simulink model "cornering_simulation_self_contained"  (R2026a)
settings: Solver=VariableStepAuto
settings Model: Creator=mattr  LastModifiedBy=mattr

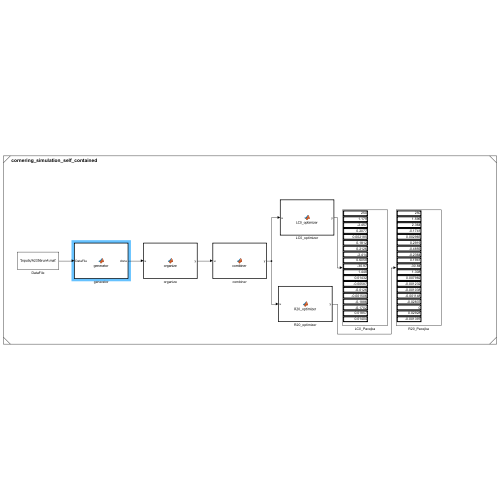
[thumbnail: Simulink's stored preview of the top-level diagram]
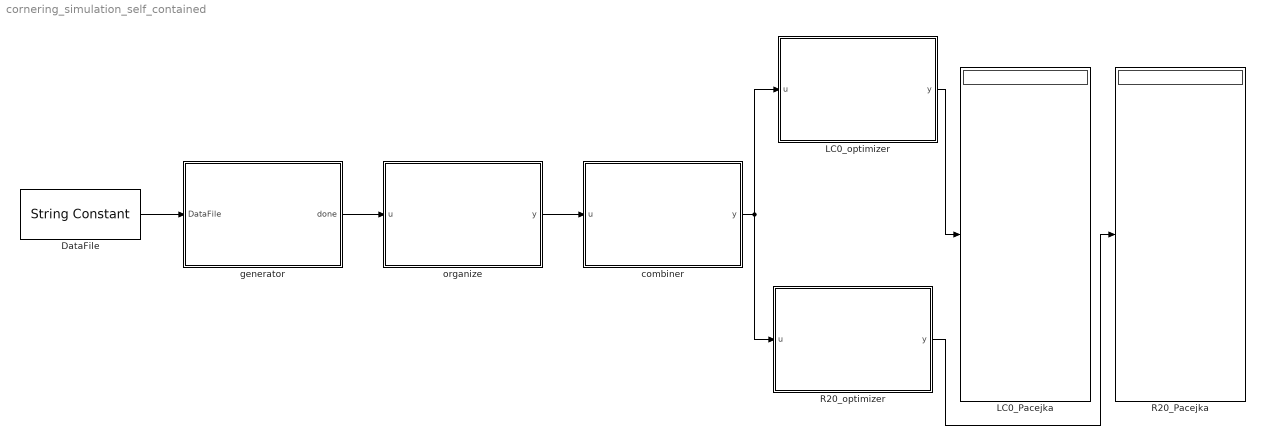
== system cornering_simulation_self_contained ==
  DataFile : StringConstant  String='Inputs/A2356run4.mat'
  LC0_Pacejka : Display
  LC0_optimizer : MATLAB Function  TreatAsAtomicUnit=on
  R20_Pacejka : Display
  R20_optimizer : MATLAB Function  TreatAsAtomicUnit=on
  combiner : MATLAB Function  TreatAsAtomicUnit=on
  generator : MATLAB Function  TreatAsAtomicUnit=on
  organize : MATLAB Function  TreatAsAtomicUnit=on
  wires:
  organize/1(y) -> combiner/1(u)
  combiner/1(y) -> R20_optimizer/1(u), LC0_optimizer/1(u)
  generator/1(done) -> organize/1(u)
  R20_optimizer/1(y) -> R20_Pacejka/1
  LC0_optimizer/1(y) -> LC0_Pacejka/1
  DataFile/1 -> generator/1(DataFile)

== matlab function cornering_simulation_self_contained/generator ==
  data: DataFile input; done output
function done = generator(DataFile)
    coder.extrinsic('evalin', 'assignin', 'disp');
    
    done = 0;
    persistent hasExecuted;
    if isempty(hasExecuted)
        hasExecuted = false;
    end
    
    if ~hasExecuted
        if isstring(DataFile)
            dataFileStr = char(DataFile);
        elseif ischar(DataFile)
            dataFileStr = DataFile;
        else
            dataFileStr = char(DataFile(:)');
        end
        
        assignin('base', 'gen_dataFileStr', dataFileStr);
        evalin('base', [ ...
            'outputFolder = ''data/Outputs/R20Round4&5''; ' ...
            'if ~exist(outputFolder, ''dir''), mkdir(outputFolder); end; ' ...
            'curFile = load(gen_dataFileStr); ' ...
            'disp(["Loaded " gen_dataFileStr]); ' ...
            'runTable = table(curFile.AMBTMP, curFile.ET, curFile.FX, curFile.FY, curFile.FZ, curFile.IA, curFile.MX, curFile.MZ, ' ...
            'curFile.N, curFile.NFX, curFile.NFY, curFile.P, curFile.RE, curFile.RL, curFile.RST, ' ...
            'curFile.SA, curFile.SL, curFile.SR, curFile.TSTC, curFile.TSTI, curFile.TSTO, curFile.V, ' ...
            '''VariableNames'', {''AmbientRoomTemperature'', ''ElapsedTime'', ''LongitudinalForce'', ''LateralForce'', ' ...
            '''NormalForce'', ''InclinationAngle'', ''OverturningMoment'', ''AligningTorque'', ''WheelRotationalSpeed'', ' ...
            '''NormalizedLongitudinalForce_FX_FZ'', ''NormalizedLateralForce_FY_FZ'', ''TirePressure'', ' ...
            '''EffectiveRadius'', ''LoadedRadius'', ''RoadSurfaceTemperature'', ''SlipAngle'', ''SlipRatioTextbook'', ' ...
            '''SlipRatioBasedOnRL'', ''TireSurfaceTemperature_Center'', ''TireSurfaceTemperature_Inboard'', ' ...
            '''TireSurfaceTemperature_Outboard'', ''RoadSpeed''}); ' ...
            'runTable.testid = repmat(string(curFile.testid), height(runTable), 1); ' ...
            'runTable.tireid = repmat(string(curFile.tireid), height(runTable), 1); ' ...
            'runTable.Index = (1:height(runTable))''; ' ...
            'nRows = height(runTable); ' ...
            'subTables = struct(); ' ...
            'subTables.FZ50  = runTable(5006:min(6220, nRows), :); ' ...
            'subTables.FZ100 = runTable(7491:min(8645, nRows), :); ' ...
            'subTables.FZ150 = runTable(3754:min(4937, nRows), :); ' ...
            'subTables.FZ200 = runTable(2546:min(3667, nRows), :); ' ...
            'subTables.FZ250 = [runTable(1:min(2484, nRows), :); runTable(6255:min(7418, nRows), :)]; ' ...
            'outNames = fieldnames(subTables); ' ...
            'for i = 1:numel(outNames) ' ...
            '    fname = fullfile(outputFolder, sprintf("R20_FZ_%s.csv", outNames{i}(3:end))); ' ...
            '    writetable(subTables.(outNames{i}), fname); ' ...
            '    disp(["Saved: " fname]); ' ...
            'end; ' ...
            'disp("All FZ bin CSV files successfully exported.");' ...
        ]);
        
        hasExecuted = true;
    end
    
    done = 1;
end

%% Here is the code as it should be commented above

% function generator()
%
%dataFile     = 'Inputs/A2356run4.mat';     % Change this to round you want
%outputFolder = 'data/Outputs/R20Round4&5'; % Change this to output you want
%
%%% Ensure the output folder exists
%if ~exist(outputFolder, 'dir')
%    mkdir(outputFolder)
%end
%
%% Change these based off of inclination angle/tire type (see Teams)
%idxRange50   = 5006:6220;
%idxRange100  = 7491:8645;
%idxRange150  = 3754:4937;
%idxRange200  = 2546:3667;
%idxRange250a = 1:2484;
%idxRange250b = 6255:7418;

%curFile = load(dataFile);
%disp("Loaded " + dataFile);

%%% Create the table and give names to each of the variables
%runTable = table(curFile.AMBTMP, curFile.ET, curFile.FX, curFile.FY, curFile.FZ, curFile.IA, curFile.MX, curFile.MZ, ...
%    curFile.N, curFile.NFX, curFile.NFY, curFile.P, curFile.RE, curFile.RL, curFile.RST, ...
%    curFile.SA, curFile.SL, curFile.SR, curFile.TSTC, curFile.TSTI, curFile.TSTO, curFile.V, ...
%    'VariableNames', {'AmbientRoomTemperature', 'ElapsedTime', 'LongitudinalForce', 'LateralForce', ...
%    'NormalForce', 'InclinationAngle', 'OverturningMoment', 'AligningTorque', 'WheelRotationalSpeed', ...
%    'NormalizedLongitudinalForce(FX/FZ)', 'NormalizedLateralForce(FY/FZ)', 'TirePressure', ...
%    'EffectiveRadius', 'LoadedRadius', 'RoadSurfaceTemperature', 'SlipAngle', 'SlipRatioTextbook', ...
%    'SlipRatioBasedOnRL', 'TireSurfaceTemperature-Center', 'TireSurfaceTemperature-Inboard', ...
%    'TireSurfaceTemperature-Outboard', 'RoadSpeed'});


%%% Ensure every row has the testid and tireid 
%runTable.testid = repmat(string(curFile.testid), height(runTable), 1);
%runTable.tireid = repmat(string(curFile.tireid), height(runTable), 1);

%%% Index column updated to count up by row starting at 1
%runTable.Index = (1:height(runTable))';

%disp("Run table created with " + height(runTable) + " rows.");

%subTables = struct();

%%% Extracts sub tables from runTable based on the ranges set above
%subTables.FZ50  = runTable(idxRange50,  :);
%subTables.FZ100 = runTable(idxRange100, :);
%subTables.FZ150 = runTable(idxRange150, :);
%subTables.FZ200 = runTable(idxRange200, :);
%subTables.FZ250 = [runTable(idxRange250a, :); runTable(idxRange250b, :)];

%%% Names of all of the FZs 
%outNames = fieldnames(subTables);

%%% Generate output files into the output folder with a naming scheme
%for i = 1:numel(outNames)
%    fname = fullfile(outputFolder, sprintf("R20_FZ_%s.csv", outNames{i}(3:end))); % Change this for tire type/inclination angle
%    writetable(subTables.(outNames{i}), fname);
%    disp("Saved: " + fname);
%end

%disp("All FZ bin CSV files successfully exported.");

%end

== matlab function cornering_simulation_self_contained/combiner ==
  data: u input; y output
function y = combiner(u)
    coder.extrinsic('evalin', 'disp');
    
    y = 0;
    persistent hasExecuted;
    if isempty(hasExecuted)
        hasExecuted = false;
    end
    
    if (u > 0)
        if ~hasExecuted
            evalin('base', [ ...
                'dataFolder = ''data/Outputs/R20Round4&5''; ' ...
                'filteredFiles = dir(fullfile(dataFolder, ''*_filtered.csv'')); ' ...
                'combinedTable = table(); ' ...
                'for i = 1:numel(filteredFiles) ' ...
                '    if contains(filteredFiles(i).name, "combined"), continue; end; ' ...
                '    curFile = fullfile(filteredFiles(i).folder, filteredFiles(i).name); ' ...
                '    disp(["Adding " filteredFiles(i).name]); ' ...
                '    tempTable = readtable(curFile); ' ...
                '    [~, name, ~] = fileparts(filteredFiles(i).name); ' ...
                '    tempTable.SourceFile = repmat({name}, height(tempTable), 1); ' ...
                '    combinedTable = [combinedTable; tempTable]; ' ...
                'end; ' ...
                'combinedTable = sortrows(combinedTable, ''NormalForce''); ' ...
                'outPath = fullfile(dataFolder, ''R20_combined_filtered.csv''); ' ...
                'writetable(combinedTable, outPath); ' ...
                'disp(["Combined filtered data saved as: " outPath]);' ...
            ]);
            hasExecuted = true;
        end
        y = 1;
    end
end

%% Here is the code as it should be commented 

%function combiner()
% 
%     dataFolder = 'data/Outputs/R20Round4&5';
% 
%     %% All of the files from organize.m
%     filteredFiles = dir(fullfile(dataFolder, '*_filtered.csv'));
% 
%     combinedTable = table();
% 
%     for i = 1:numel(filteredFiles)
%         curFile = fullfile(filteredFiles(i).folder, filteredFiles(i).name);
%         disp("Adding " + filteredFiles(i).name);
% 
%         tempTable = readtable(curFile);
% 
%         [~, name, ~] = fileparts(filteredFiles(i).name);
%         tempTable.SourceFile = repmat({name}, height(tempTable), 1);
% 
%         combinedTable = [combinedTable; tempTable];
%     end
% 
%     combinedTable = sortrows(combinedTable, 'NormalForce');
% 
%     outPath = fullfile(dataFolder, 'R20_combined_filtered.csv');
%     writetable(combinedTable, outPath);
% 
%     disp("Combined filtered data saved as: " + outPath);
% 
% 
% end

== matlab function cornering_simulation_self_contained/LC0_optimizer ==
  data: u input; y output size=[19 1]
function y = LC0_optimizer(u)
    coder.extrinsic('evalin', 'disp');
    
    y = zeros(19, 1);
    
    persistent hasExecuted;
    if isempty(hasExecuted)
        hasExecuted = false;
    end
    
    if (u > 0)
        if ~hasExecuted
            evalin('base', [ ...
                'pacejka_calc = @(P, L, FZ, IA, alpha) (' ...
                '    (FZ .* (P(3) + P(4) * ((FZ - P(1)) / P(1))) .* (1 - P(5) * IA.^2) * L(1)) .* ' ...
                '    sin((P(2) * L(2)) * atan(' ...
                '        (((P(10) * P(1) * sin(2 * atan(FZ / (P(11) * P(1) * L(3))))) .* (1 - P(12) * abs(IA)) * L(4) * L(5)) ./ ' ...
                '        ((P(2) * L(2)) * (FZ .* (P(3) + P(4) * ((FZ - P(1)) / P(1))) .* (1 - P(5) * IA.^2) * L(1)))) .* ' ...
                '        (alpha + (P(13) + P(14) * ((FZ - P(1)) / P(1)) + P(15) * IA) * L(6)) - ' ...
                '        ((P(6) + P(7) * ((FZ - P(1)) / P(1))) .* (1 - (P(8) + P(9) * IA) .* sign(alpha)) * L(7)) .* ' ...
                '        (' ...
                '            (((P(10) * P(1) * sin(2 * atan(FZ / (P(11) * P(1) * L(3))))) .* (1 - P(12) * abs(IA)) * L(4) * L(5)) ./ ' ...
                '            ((P(2) * L(2)) * (FZ .* (P(3) + P(4) * ((FZ - P(1)) / P(1))) .* (1 - P(5) * IA.^2) * L(1)))) .* ' ...
                '            (alpha + (P(13) + P(14) * ((FZ - P(1)) / P(1)) + P(15) * IA) * L(6)) - ' ...
                '            atan(' ...
                '                (((P(10) * P(1) * sin(2 * atan(FZ / (P(11) * P(1) * L(3))))) .* (1 - P(12) * abs(IA)) * L(4) * L(5)) ./ ' ...
                '                ((P(2) * L(2)) * (FZ .* (P(3) + P(4) * ((FZ - P(1)) / P(1))) .* (1 - P(5) * IA.^2) * L(1)))) .* ' ...
                '                (alpha + (P(13) + P(14) * ((FZ - P(1)) / P(1)) + P(15) * IA) * L(6))' ...
                '            )' ...
                '        )' ...
                '    )) + FZ .* (P(16) + P(17) * ((FZ - P(1)) / P(1)) + (P(18) + P(19) * ((FZ - P(1)) / P(1))) .* IA) * L(8) * L(5)' ...
                '); ' ...
                'files = {''data/LC0_combined_filtered.csv'', ''data/LC0_IA-2_combined_filtered.csv'', ''data/LC0_IA-4_combined_filtered.csv''}; ' ...
                'validFiles = files(cellfun(@(f) exist(f, ''file'') > 0, files)); ' ...
                'if isempty(validFiles), disp(''Warning: LC0 CSV input files not found. Returning baseline P0.''); LC0_opt_y = [250, 1.17858, -2.45689, 0.207723, 0.00218554, 0.181269, 0.212474, -2.41388, 0.605724, -30.9683, 1.44763, 0.0143188, -0.00587066, -0.0126017, -0.00150596, -0.18861, -0.170156, 0.0185739, 0.0140275]''; else ' ...
                'data = []; for k = 1:numel(validFiles), data = [data; readtable(validFiles{k})]; end; ' ...
                'IA = data.InclinationAngle; FZRaw = data.NormalForce; alpha = data.SlipAngle; FYExperimental = data.LateralForce; source = data.SourceFile; ' ...
                'FZBins = [50, 100, 150, 200, 250]; FYAll = []; FZAll = []; alphaAll = []; IAAll = []; ' ...
                'for i = 1:numel(FZBins), baseTag = sprintf(''LC0_FZ_%d'', FZBins(i)); idx = contains(source, [baseTag ''_filtered'']) | contains(source, [baseTag ''_IA-2_filtered'']) | contains(source, [baseTag ''_IA-4_filtered'']); FYAll = [FYAll; FYExperimental(idx)]; FZAll = [FZAll; FZBins(i) * ones(sum(idx),1)]; alphaAll = [alphaAll; alpha(idx)]; IAAll = [IAAll; IA(idx)]; end; ' ...
                'alphaAll = deg2rad(alphaAll); ' ...
                'P0 = [250, 1.17858, -2.45689, 0.207723, 0.00218554, 0.181269, 0.212474, -2.41388, 0.605724, -30.9683, 1.44763, 0.0143188, -0.00587066, -0.0126017, -0.00150596, -0.18861, -0.170156, 0.0185739, 0.0140275]; ' ...
                'L = ones(1,8); ' ...
                'w_vec = zeros(size(IAAll)); IAvals = unique(IAAll); ' ...
                'for k = 1:numel(IAvals), idx = (IAAll == IAvals(k)); w_vec(idx) = 1 / max(sum(idx), 1); end; ' ...
                'options = optimoptions(''lsqnonlin'', ''Display'', ''iter'', ''MaxFunctionEvaluations'', 20000, ''TolFun'', 1e-8, ''TolX'', 1e-8); ' ...
                'lb = -Inf(1,19); ub = Inf(1,19); lb(1) = 250; ub(1) = 250; ' ...
                'POptimization = lsqnonlin(@(P) w_vec .* (pacejka_calc(P, L, FZAll, IAAll, alphaAll) - FYAll), P0, lb, ub, options); ' ...
                'LC0_opt_y = POptimization(:); disp(''LC0 Optimized Parameters:''); disp(LC0_opt_y); ' ...
                'IAValues = unique(IAAll); colors = lines(numel(FZBins)); ' ...
                'for k = 1:numel(IAValues) ' ...
                '    thisIA = IAValues(k); fig = figure(''Name'', sprintf(''LC0 Pacejka Fit - IA = %.1f deg'', thisIA), ''Visible'', ''on''); hold on; grid on; ' ...
                '    idxIA = (IAAll == thisIA); ' ...
                '    for i = 1:numel(FZBins) ' ...
                '        idx = idxIA & (FZAll == FZBins(i)); ' ...
                '        if any(idx) ' ...
                '            scatter(rad2deg(alphaAll(idx)), FYAll(idx), 10, colors(i,:), ''filled'', ''DisplayName'', sprintf(''Exp FZ=%d'', FZBins(i))); ' ...
                '            [alphaSort, ~] = sort(alphaAll(idx)); ' ...
                '            FYFit = pacejka_calc(POptimization, L, FZAll(idx), IAAll(idx), alphaSort); ' ...
                '            plot(rad2deg(alphaSort), FYFit, ''Color'', colors(i,:), ''LineWidth'', 1.5, ''DisplayName'', sprintf(''Fit FZ=%d'', FZBins(i))); ' ...
                '        end; ' ...
                '    end; ' ...
                '    title(sprintf(''LC0 Pacejka Fit - IA = %.1f deg'', thisIA)); xlabel(''Slip Angle [deg]''); ylabel(''Lateral Force FY [N]''); legend(''Location'', ''best''); ' ...
                '    saveas(fig, sprintf(''data/Outputs/R20Round4&5/LC0_Pacejka_Fit_IA_%.0f.png'', thisIA)); drawnow; ' ...
                'end; end;' ...
            ]);
            hasExecuted = true;
        end
        
        y_temp = evalin('base', 'LC0_opt_y');
        y(:) = y_temp;
    end
end

%% Here is the code as it should be commented 

% function POptimization = LC0_optimizer()
% 
%     data0 = readtable('data/LC0_combined_filtered.csv');
%     data2 = readtable('data/LC0_IA-2_combined_filtered.csv');
%     data4 = readtable('data/LC0_IA-4_combined_filtered.csv');
%     data  = [data0; data2; data4;];
% 
%     % Column meanings
%     IA             = data.InclinationAngle;  % Inclination angle (held constant at 0)
%     FZRaw          = data.NormalForce;       % Normal force
%     alpha          = data.SlipAngle;         % Slip angle (deg)
%     FYExperimental = data.LateralForce;      % Experimental lateral force
%     source         = data.SourceFile;        % Source file name
% 
%     FZBins   = [50, 100, 150, 200, 250];
%     FYAll    = [];
%     FZAll    = [];
%     alphaAll = [];
%     IAAll    = [];
% 
%     for i = 1:numel(FZBins)
%         baseTag = sprintf('LC0_FZ_%d', FZBins(i));
% 
%         % Match any of these forms:
%         % R20_FZ_*_filtered
%         % R20_FZ_*_IA-2_filtered
%         % R20_FZ_*_IA-4_filtered
%         % Also works for LC0 just match format for new tire
%         idx = contains(source, [baseTag '_filtered']) | contains(source, [baseTag '_IA-2_filtered']) | contains(source, [baseTag '_IA-4_filtered']);
% 
%         FYAll    = [FYAll; FYExperimental(idx)];
%         FZAll    = [FZAll; FZBins(i) * ones(sum(idx),1)];
%         alphaAll = [alphaAll; alpha(idx)];
%         IAAll    = [IAAll; IA(idx)];
%     end
% 
%     alphaAll = deg2rad(alphaAll);
% 
%     P0 = [250, 1.17858, -2.45689, 0.207723, 0.00218554, 0.181269, 0.212474, -2.41388, 0.605724, -30.9683, 1.44763, 0.0143188, -0.00587066, -0.0126017, -0.00150596, -0.18861, -0.170156, 0.0185739, 0.0140275];
%     L = ones(1,8);
% 
%     objFun = @(P) FYExperimental_all(P, L, FZAll, IAAll, alphaAll, FYAll);
% 
%     %options = optimoptions('lsqnonlin','Display', 'iter', 'MaxFunctionEvaluations', 40000, 'TolFun', 1e-10, 'TolX', 1e-10, 'UseParallel', true);
% 
%     options = optimoptions('lsqnonlin', 'Display', 'iter', 'MaxFunctionEvaluations', 20000, 'TolFun', 1e-8, 'TolX', 1e-8);
% 
%     lb = -Inf(1,19);
%     ub = Inf(1,19);
%     % Fix PEY2, PEY3, PEY4, PHY2, PVY2 to zero
%     %fixedIdx = [2, 3, 6, 4, 10, 11, 12]; % Parameter positions to fix
%     %fixedZeroes = [8, 9, 13, 17, 18]
%     lb(1) = 250;
%     ub(1) = 250;
%     %lb(fixedIdx) = P0(fixedIdx);
%     %ub(fixedIdx) = P0(fixedIdx);
%     %lb(fixedZeroes) = 0;
%     %ub(fixedZeroes) = 0;
% 
%     POptimization = lsqnonlin(objFun, P0, lb, ub, options);
%     POptimization = POptimization(:); % Convert row to column vector
%     disp('Optimized Parameters:')
%     disp(POptimization)
% 
%     FYPredicted = pacejka(POptimization, L, FZAll, IAAll, alphaAll);
%     rmse = sqrt(mean((FYAll - FYPredicted).^2));
%     fprintf('Overall RMSE: %.3f\n', rmse);
% 
% 
%     IAValues = [0, 2, 4];
%     colors = lines(numel(FZBins));
% 
%     for k = 1:numel(IAValues)
%         fig = figure('Visible', 'on', 'Name', sprintf('LC0 Pacejka Fit - IA = %d°', IAValues(k)));
%         hold on;
%         grid on;
%         thisIA = IAValues(k);
%         idxIA = (IAAll == thisIA);
% 
%         for i = 1:numel(FZBins)
%             idx = idxIA & (FZAll == FZBins(i));
%             scatter(rad2deg(alphaAll(idx)), FYAll(idx), 2, colors(i,:), 'filled', 'DisplayName', sprintf('Exp FZ=%d', FZBins(i)));
%             [alphaSort, ~] = sort(alphaAll(idx));
%             FYFit = pacejka(POptimization, L, FZAll(idx), IAAll(idx), alphaSort);
%             plot(rad2deg(alphaSort), FYFit, 'Color', colors(i,:), 'LineWidth', 1.5, 'DisplayName', sprintf('Fit FZ=%d', FZBins(i)));
%         end
% 
%         title(sprintf('Pacejka Fit - IA = %d° (RMSE = %.2f)', thisIA, rmse));
%         xlabel('Slip Angle [deg]');
%         ylabel('Lateral Force FY');
%         legend('Location', 'best');
% 
%         saveas(fig, sprintf('data/Outputs/LC0_Pacejka_Fit_IA_%d.png', thisIA));
% 
%         drawnow; 
%     end
% 
% 
% end
% 
% function err = FYExperimental_all(P, L, FZ, IA, alpha, FYExperimental)
%     FYModel = pacejka(P, L, FZ, IA, alpha);
% 
%     % Weight residuals so each inclination angle (IA) contributes equally
%     IAvals = unique(IA);
%     err = [];
%     for i = 1:numel(IAvals)
%         idx = IA == IAvals(i);
%         n = sum(idx);
%         w = 1 / max(n, 1);  % equal total contribution per IA group
%         err = [err; w * (FYModel(idx) - FYExperimental(idx))];
%     end
% end

== matlab function cornering_simulation_self_contained/R20_optimizer ==
  data: u input; y output size=[19 1]
function y = R20_optimizer(u)
    coder.extrinsic('evalin', 'disp');
    
    y = zeros(19, 1);
    
    persistent hasExecuted;
    if isempty(hasExecuted)
        hasExecuted = false;
    end
    
    if (u > 0)
        if ~hasExecuted
            evalin('base', [ ...
                'pacejka_calc = @(P, L, FZ, IA, alpha) (' ...
                '    (FZ .* (P(3) + P(4) * ((FZ - P(1)) / P(1))) .* (1 - P(5) * IA.^2) * L(1)) .* ' ...
                '    sin((P(2) * L(2)) * atan(' ...
                '        (((P(10) * P(1) * sin(2 * atan(FZ / (P(11) * P(1) * L(3))))) .* (1 - P(12) * abs(IA)) * L(4) * L(5)) ./ ' ...
                '        ((P(2) * L(2)) * (FZ .* (P(3) + P(4) * ((FZ - P(1)) / P(1))) .* (1 - P(5) * IA.^2) * L(1)))) .* ' ...
                '        (alpha + (P(13) + P(14) * ((FZ - P(1)) / P(1)) + P(15) * IA) * L(6)) - ' ...
                '        ((P(6) + P(7) * ((FZ - P(1)) / P(1))) .* (1 - (P(8) + P(9) * IA) .* sign(alpha)) * L(7)) .* ' ...
                '        (' ...
                '            (((P(10) * P(1) * sin(2 * atan(FZ / (P(11) * P(1) * L(3))))) .* (1 - P(12) * abs(IA)) * L(4) * L(5)) ./ ' ...
                '            ((P(2) * L(2)) * (FZ .* (P(3) + P(4) * ((FZ - P(1)) / P(1))) .* (1 - P(5) * IA.^2) * L(1)))) .* ' ...
                '            (alpha + (P(13) + P(14) * ((FZ - P(1)) / P(1)) + P(15) * IA) * L(6)) - ' ...
                '            atan(' ...
                '                (((P(10) * P(1) * sin(2 * atan(FZ / (P(11) * P(1) * L(3))))) .* (1 - P(12) * abs(IA)) * L(4) * L(5)) ./ ' ...
                '                ((P(2) * L(2)) * (FZ .* (P(3) + P(4) * ((FZ - P(1)) / P(1))) .* (1 - P(5) * IA.^2) * L(1)))) .* ' ...
                '                (alpha + (P(13) + P(14) * ((FZ - P(1)) / P(1)) + P(15) * IA) * L(6))' ...
                '            )' ...
                '        )' ...
                '    )) + FZ .* (P(16) + P(17) * ((FZ - P(1)) / P(1)) + (P(18) + P(19) * ((FZ - P(1)) / P(1))) .* IA) * L(8) * L(5)' ...
                '); ' ...
                'files = {''data/Outputs/R20Round4&5/R20_combined_filtered.csv'', ''data/R20_IA-2_combined_filtered.csv'', ''data/R20_IA-4_combined_filtered.csv''}; ' ...
                'validFiles = files(cellfun(@(f) exist(f, ''file'') > 0, files)); ' ...
                'if isempty(validFiles), disp(''Warning: R20 CSV input files not found. Returning baseline P0.''); R20_opt_y = [250, 1.4, 2.4, -0.25, 3, -0.1, -1.5, 0, 0, -30.5, 1.15, 1, 0, 0, -0.128, 0, 0, 0, 1.43]''; else ' ...
                'data = []; for k = 1:numel(validFiles), data = [data; readtable(validFiles{k})]; end; ' ...
                'IA = data.InclinationAngle; FZRaw = data.NormalForce; alpha = data.SlipAngle; FYExperimental = data.LateralForce; source = data.SourceFile; ' ...
                'FZBins = [50, 100, 150, 200, 250]; FYAll = []; FZAll = []; alphaAll = []; IAAll = []; ' ...
                'for i = 1:numel(FZBins), baseTag = sprintf(''R20_FZ_%d'', FZBins(i)); idx = contains(source, [baseTag ''_filtered'']) | contains(source, [baseTag ''_IA-2_filtered'']) | contains(source, [baseTag ''_IA-4_filtered'']); FYAll = [FYAll; FYExperimental(idx)]; FZAll = [FZAll; FZBins(i) * ones(sum(idx),1)]; alphaAll = [alphaAll; alpha(idx)]; IAAll = [IAAll; IA(idx)]; end; ' ...
                'alphaAll = deg2rad(alphaAll); ' ...
                'P0 = [250, 1.4, 2.4, -0.25, 3, -0.1, -1.5, 0, 0, -30.5, 1.15, 1, 0, 0, -0.128, 0, 0, 0, 1.43]; ' ...
                'L = ones(1,8); ' ...
                'options = optimoptions(''lsqnonlin'', ''Display'', ''iter'', ''MaxFunctionEvaluations'', 20000, ''TolFun'', 1e-8, ''TolX'', 1e-8); ' ...
                'lb = -Inf(1,19); ub = Inf(1,19); fixedIdx = 17; lb(1) = 250; ub(1) = 250; lb(fixedIdx) = P0(fixedIdx); ub(fixedIdx) = P0(fixedIdx); ' ...
                'POptimization = lsqnonlin(@(P) pacejka_calc(P, L, FZAll, IAAll, alphaAll) - FYAll, P0, lb, ub, options); ' ...
                'R20_opt_y = POptimization(:); disp(''R20 Optimized Parameters:''); disp(R20_opt_y); ' ...
                'IAValues = unique(IAAll); colors = lines(numel(FZBins)); ' ...
                'for k = 1:numel(IAValues) ' ...
                '    thisIA = IAValues(k); fig = figure(''Name'', sprintf(''R20 Pacejka Fit - IA = %.1f deg'', thisIA), ''Visible'', ''on''); hold on; grid on; ' ...
                '    idxIA = (IAAll == thisIA); ' ...
                '    for i = 1:numel(FZBins) ' ...
                '        idx = idxIA & (FZAll == FZBins(i)); ' ...
                '        if any(idx) ' ...
                '            scatter(rad2deg(alphaAll(idx)), FYAll(idx), 10, colors(i,:), ''filled'', ''DisplayName'', sprintf(''Exp FZ=%d'', FZBins(i))); ' ...
                '            [alphaSort, ~] = sort(alphaAll(idx)); ' ...
                '            FYFit = pacejka_calc(POptimization, L, FZAll(idx), IAAll(idx), alphaSort); ' ...
                '            plot(rad2deg(alphaSort), FYFit, ''Color'', colors(i,:), ''LineWidth'', 1.5, ''DisplayName'', sprintf(''Fit FZ=%d'', FZBins(i))); ' ...
                '        end; ' ...
                '    end; ' ...
                '    title(sprintf(''R20 Pacejka Fit - IA = %.1f deg'', thisIA)); xlabel(''Slip Angle [deg]''); ylabel(''Lateral Force FY [N]''); legend(''Location'', ''best''); ' ...
                '    saveas(fig, sprintf(''data/Outputs/R20Round4&5/R20_Pacejka_Fit_IA_%.0f.png'', thisIA)); drawnow; ' ...
                'end; end;' ...
            ]);
            hasExecuted = true;
        end
        
        y_temp = evalin('base', 'R20_opt_y');
        y(:) = y_temp;
    end
end

%% Here is the code as it should be commented

% function POptimization = R20_optimizer()
% 
%     data0 = readtable('data/R20_combined_filtered.csv');
%     data2 = readtable('data/R20_IA-2_combined_filtered.csv');
%     data4 = readtable('data/R20_IA-4_combined_filtered.csv');
%     data = [data0; data2; data4];
% 
%     % Column meanings
%     IA             = data.InclinationAngle;  % Inclination angle (held constant at 0)
%     FZRaw          = data.NormalForce;       % Normal force
%     alpha          = data.SlipAngle;         % Slip angle (deg)
%     FYExperimental = data.LateralForce;      % Experimental lateral force
%     source         = data.SourceFile;        % Source file name
% 
%     FZBins   = [50, 100, 150, 200, 250];
%     FYAll    = [];
%     FZAll    = [];
%     alphaAll = [];
%     IAAll    = [];
% 
%     for i = 1:numel(FZBins)
%         baseTag = sprintf('R20_FZ_%d', FZBins(i));
% 
%         % Match any of these forms:
%         % R20_FZ_*_filtered
%         % R20_FZ_*_IA-2_filtered
%         % R20_FZ_*_IA-4_filtered
%         idx = contains(source, [baseTag '_filtered']) | contains(source, [baseTag '_IA-2_filtered']) | contains(source, [baseTag '_IA-4_filtered']);
% 
%         FYAll    = [FYAll; FYExperimental(idx)];
%         FZAll    = [FZAll; FZBins(i) * ones(sum(idx),1)];
%         alphaAll = [alphaAll; alpha(idx)];
%         IAAll    = [IAAll; IA(idx)];
%     end
% 
%     alphaAll = deg2rad(alphaAll);
% 
%     P0 = [250, 1.4, 2.4, -0.25, 3, -0.1, -1.5, 0, 0, -30.5, 1.15, 1, 0, 0, -0.128, 0, 0, 0, 1.43];
%     L  = ones(1,8);
% 
%     objFun = @(P) FYExperimental_all(P, L, FZAll, IAAll, alphaAll, FYAll);
% 
%     options = optimoptions('lsqnonlin', 'Display', 'iter', 'MaxFunctionEvaluations', 20000, 'TolFun', 1e-8, 'TolX', 1e-8);
% 
%     lb = -Inf(1,19);
%     ub = Inf(1,19);
%     % Fix PEY2, PEY3, PEY4, PHY2, PVY2 to zero
%     fixedIdx = [17]; % Parameter positions to fix
%     lb(1) = 250;
%     ub(1) = 250;
%     lb(fixedIdx) = P0(fixedIdx);
%     ub(fixedIdx) = P0(fixedIdx);
% 
% 
%     POptimization = lsqnonlin(objFun, P0, lb, ub, options);
%     POptimization = POptimization(:); % Convert row to column vector
%     disp('Optimized Parameters:')
%     disp(POptimization)
% 
%     FYPredicted = pacejka(POptimization, L, FZAll, IAAll, alphaAll);
%     rmse = sqrt(mean((FYAll - FYPredicted).^2));
%     fprintf('Overall RMSE: %.3f\n', rmse);
% 
% 
%     IAValues = [0, 2, 4];
%     colors = lines(numel(FZBins));
% 
%     for k = 1:numel(IAValues)
%         fig = figure('Visible', 'on', 'Name', sprintf('R20 Pacejka Fit - IA = %d°', IAValues(k)));
%         hold on;
%         grid on;
%         thisIA = IAValues(k);
%         idxIA = (IAAll == thisIA);
% 
%         for i = 1:numel(FZBins)
%             idx = idxIA & (FZAll == FZBins(i));
%             scatter(rad2deg(alphaAll(idx)), FYAll(idx), 2, colors(i,:), 'filled', 'DisplayName', sprintf('Exp FZ=%d', FZBins(i)));
%             [alphaSort, ~] = sort(alphaAll(idx));
%             FYFit = pacejka(POptimization, L, FZAll(idx), IAAll(idx), alphaSort);
%             plot(rad2deg(alphaSort), FYFit, 'Color', colors(i,:), 'LineWidth', 1.5, 'DisplayName', sprintf('Fit FZ=%d', FZBins(i)));
%         end
% 
%         title(sprintf('Pacejka Fit - IA = %d° (RMSE = %.2f)', thisIA, rmse));
%         xlabel('Slip Angle [deg]');
%         ylabel('Lateral Force FY');
%         legend('Location', 'best');
% 
%         saveas(fig, sprintf('data/Outputs/LC0_Pacejka_Fit_IA_%d.png', thisIA));
% 
%         drawnow; 
%     end
% end
% 
% function err = FYExperimental_all(P, L, FZ, IA, alpha, FYExperimental)
%     FYModel = pacejka(P, L, FZ, IA, alpha);
%     err = FYModel - FYExperimental;   % residuals for lsqnonlin
% end

== matlab function cornering_simulation_self_contained/organize ==
  data: u input; y output
function y = organize(u)
    coder.extrinsic('evalin', 'disp');
    
    y = 0;
    persistent hasExecuted;
    if isempty(hasExecuted)
        hasExecuted = false;
    end
    
    if (u > 0)
        if ~hasExecuted
            evalin('base', [ ...
                'dataFolder = ''data/Outputs/R20Round4&5''; ' ...
                'csvFiles = dir(fullfile(dataFolder, "R20_FZ_*.csv")); ' ...
                'for i = 1:numel(csvFiles) ' ...
                '    if contains(csvFiles(i).name, "_filtered"), continue; end; ' ...
                '    curFile = fullfile(csvFiles(i).folder, csvFiles(i).name); ' ...
                '    disp(["Processing " csvFiles(i).name]); ' ...
                '    tbl = readtable(curFile); ' ...
                '    varNames = ["RoadSpeed", "TirePressure", "InclinationAngle", "NormalForce", "SlipAngle", "ElapsedTime", "LateralForce", "Index"]; ' ...
                '    tbl = tbl(:, varNames); ' ...
                '    tbl.RoadSpeed        = round(tbl.RoadSpeed); ' ...
                '    tbl.TirePressure     = floor(tbl.TirePressure); ' ...
                '    tbl.InclinationAngle = floor(tbl.InclinationAngle * 10) / 10; ' ...
                '    tbl = sortrows(tbl, ["RoadSpeed", "TirePressure", "InclinationAngle"]); ' ...
                '    filteredTable = tbl(tbl.InclinationAngle == 0 & tbl.RoadSpeed == 25 & tbl.TirePressure == 12, :); ' ...
                '    filteredTable = sortrows(filteredTable, "ElapsedTime"); ' ...
                '    [~, name, ~] = fileparts(csvFiles(i).name); ' ...
                '    outName = sprintf(''%s_filtered.csv'', name); ' ...
                '    outPath = fullfile(dataFolder, outName); ' ...
                '    writetable(filteredTable, outPath); ' ...
                '    disp(["Saved filtered version: " outName]); ' ...
                '    fig = figure(''Name'', outName, ''NumberTitle'', ''off'', ''Visible'', ''off''); ' ...
                '    t  = filteredTable.ElapsedTime; ' ...
                '    NF = filteredTable.NormalForce; ' ...
                '    SA = filteredTable.SlipAngle; ' ...
                '    CF = filteredTable.LateralForce; ' ...
                '    plot(t, NF, ''b-'', ''LineWidth'', 1.5); hold on; ' ...
                '    plot(t, SA, ''r-'', ''LineWidth'', 1.5); ' ...
                '    plot(t, CF, ''g-'', ''LineWidth'', 1.5); ' ...
                '    hold off; grid on; ' ...
                '    xlabel(''Elapsed Time (s)''); ylabel(''Value''); ' ...
                '    title(strrep(outName, ''_'', ''\_'')); ' ...
                '    legend(''Normal Force (N)'', ''Slip Angle (deg)'', ''Lateral Force (N)'', ''Location'', ''best''); ' ...
                '    saveas(fig, fullfile(dataFolder, sprintf(''%s_diagnostic_plot.png'', name))); ' ...
                '    drawnow; ' ...
                '    disp(["Plot saved: " name "_diagnostic_plot.png"]); ' ...
                'end; ' ...
                'disp("All FZ bins processed, filtered, and plotted successfully.");' ...
            ]);
            hasExecuted = true;
        end
        y = 1;
    end
end

%% Here is the code as it should be commented above

% function organize()
% 
%     dataFolder = 'data/Outputs/R20Round4&5';
% 
%     %% The files generated by generate.m
%     csvFiles = dir(fullfile(dataFolder, "R20_FZ_*.csv"));
% 
%     for i = 1:numel(csvFiles)
%         if contains(csvFiles(i).name, "_filtered")
%             continue;
%         end
% 
%         curFile = fullfile(csvFiles(i).folder, csvFiles(i).name);
%         disp("Processing " + csvFiles(i).name);
% 
%         %% Extract the variables that we are interested in 
%         table = readtable(curFile);
%         varNames = ["RoadSpeed", "TirePressure", "InclinationAngle", "NormalForce", "SlipAngle", "ElapsedTime", "LateralForce", "Index"];
%         table = table(:, varNames);
% 
%         %% Normalize / round some values
%         table.RoadSpeed = round(table.RoadSpeed);
%         table.TirePressure = floor(table.TirePressure);
%         table.InclinationAngle = floor(table.InclinationAngle * 10) / 10;
% 
%         table = sortrows(table, ["RoadSpeed", "TirePressure", "InclinationAngle"]);
%         filteredTable = table(table.InclinationAngle == 0 & table.RoadSpeed == 25 & table.TirePressure == 12, :);
% 
%         filteredTable = sortrows(filteredTable, "ElapsedTime");
% 
%         [~, name, ~] = fileparts(csvFiles(i).name); %% extract just the filename (without extension)
%         outName = sprintf('%s_filtered.csv', name);
%         outPath = fullfile(dataFolder, outName);
%         writetable(filteredTable, outPath);
% 
%         disp("Saved filtered version: " + outName);
% 
%         %% Get the significant columns from the filteredTable to plot
%         figure('Name', outName, 'NumberTitle', 'off');
%         t  = filteredTable.ElapsedTime;
%         NF = filteredTable.NormalForce;
%         SA = filteredTable.SlipAngle;
%         CF = filteredTable.LateralForce;
% 
%         plot(t, NF, 'b-', 'LineWidth', 1.5); hold on;
%         plot(t, SA, 'r-', 'LineWidth', 1.5);
%         plot(t, CF, 'g-', 'LineWidth', 1.5);
%         hold off;
% 
%         grid on;
%         xlabel('Elapsed Time (s)');
%         ylabel('Value');
%         title(strrep(outName, '_', '\_'));
%         legend('Normal Force (N)', 'Slip Angle (deg)', 'Lateral Force (N)', 'Location', 'best');
% 
%         saveas(gcf, fullfile(dataFolder, sprintf('%s_diagnostic_plot.png', name)));
%         close(gcf);
% 
%         disp("Plot saved: " + name + "_diagnostic_plot.png");
%     end
% 
%     disp("All FZ bins processed, filtered, and plotted successfully.");
% 
% end
